simulink model "testModel"  (R2021b)
settings: Solver=FixedStepDiscrete  StartTime=0.0  StopTime=10.0  RelTol=1e-3
libraries: simulink x1
settings Model: DataTypeOverride=Off  Creator=tcollins  LastModifiedBy=imuthi
settings SolverCC: AlgebraicLoopSolver=TrustRegion
settings DataIOCC: LimitDataPoints=on  SaveOutput=off  SaveTime=off  ReturnWorkspaceOutputs=off
settings OptimizationCC: BlockReduction=off  ConditionallyExecuteInputs=off  DefaultParameterBehavior=Inlined  LifeSpan=inf
settings DebuggingCC: AlgebraicLoopMsg=error  SingleTaskRateTransMsg=error  AllowSymbolicDim=off  StrictBusMsg=ErrorOnBusTreatedAsVector  SFUnexpectedBacktrackingDiag=warning  SFNoUnconditionalDefaultTransitionDiag=warning  SFExecutionAtInitializationDiag=none  SFMachineParentedDataDiag=warning  ArithmeticOperatorsInVariantConditions=warning
settings HardwareCC: ProdBitPerPointer=32  ProdBitPerSizeT=32  ProdBitPerPtrDiffT=32  ProdLargestAtomicFloat=None  ProdIntDivRoundTo=Undefined  ProdEndianess=Unspecified  ProdWordSize=32  ProdHWDeviceType=ASIC/FPGA->ASIC/FPGA  ProdEqTarget=off
settings SFSimCC: SimUseLocalCustomCode=off  CustomCodeUndefinedFunction=UseInterfaceOnly
settings RTWCC: RTWUseLocalCustomCode=off
settings CodeAppCC: StateflowObjectComments=on
settings GRTTargetCC: TargetLangStandard=C89/C90 (ANSI)
settings ConfigComp: CovScope=ReferencedModels  CovMetricSettings=dw  CovSaveCumulativeToWorkspaceVar=on  CovSaveSingleToWorkspaceVar=on  CovExternalEMLEnable=off  CovSFcnEnable=off

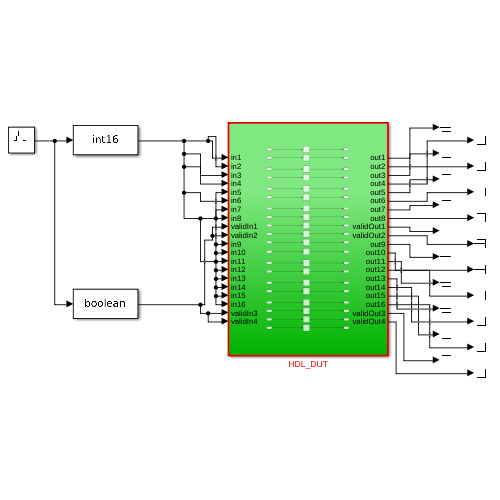
[thumbnail: Simulink's stored preview of the top-level diagram]
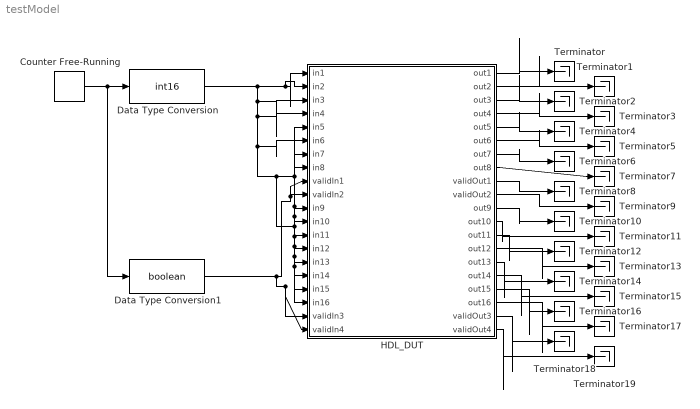
== system testModel ==
  Counter Free-Running : simulink/Sources/Counter Free-Running  NumBits=10  tsamp=1
  Data Type Conversion : DataTypeConversion  OutDataTypeStr=int16
  Data Type Conversion1 : DataTypeConversion  OutDataTypeStr=boolean
  HDL_DUT : Subsystem  TreatAsAtomicUnit=on
  Terminator{,1..19} (20 alike) : Terminator
  wires:
  Counter Free-Running/1 -> Data Type Conversion1/1, Data Type Conversion/1
  HDL_DUT/1(out1) -> Terminator/1
  HDL_DUT/2(out2) -> Terminator1/1
  HDL_DUT/3(out3) -> Terminator2/1
  HDL_DUT/4(out4) -> Terminator3/1
  Data Type Conversion/1 -> HDL_DUT/2(in2), HDL_DUT/1(in1), HDL_DUT/14(in12), HDL_DUT/16(in14), HDL_DUT/18(in16), HDL_DUT/17(in15), HDL_DUT/15(in13), HDL_DUT/11(in9), HDL_DUT/7(in7), HDL_DUT/12(in10), HDL_DUT/13(in11), HDL_DUT/5(in5), HDL_DUT/8(in8), HDL_DUT/6(in6), HDL_DUT/4(in4), HDL_DUT/3(in3)
  HDL_DUT/5(out5) -> Terminator4/1
  HDL_DUT/6(out6) -> Terminator5/1
  HDL_DUT/7(out7) -> Terminator6/1
  HDL_DUT/8(out8) -> Terminator7/1
  Data Type Conversion1/1 -> HDL_DUT/19(validIn3), HDL_DUT/20(validIn4), HDL_DUT/10(validIn2), HDL_DUT/9(validIn1)
  HDL_DUT/9(validOut1) -> Terminator8/1
  HDL_DUT/10(validOut2) -> Terminator9/1
  HDL_DUT/11(out9) -> Terminator10/1
  HDL_DUT/12(out10) -> Terminator11/1
  HDL_DUT/13(out11) -> Terminator12/1
  HDL_DUT/14(out12) -> Terminator13/1
  HDL_DUT/15(out13) -> Terminator14/1
  HDL_DUT/16(out14) -> Terminator15/1
  HDL_DUT/17(out15) -> Terminator16/1
  HDL_DUT/18(out16) -> Terminator17/1
  HDL_DUT/19(validOut3) -> Terminator18/1
  HDL_DUT/20(validOut4) -> Terminator19/1

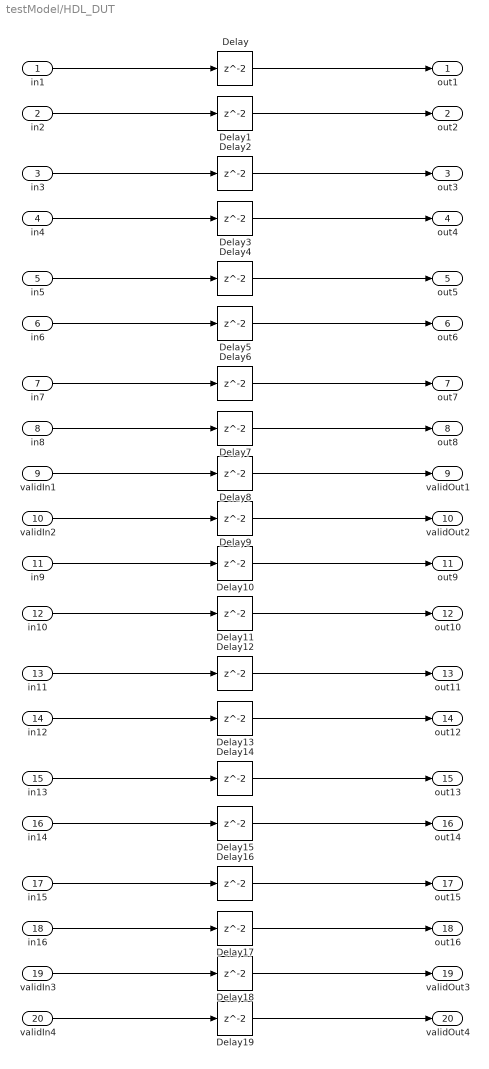
== system testModel/HDL_DUT ==
  in1 : Inport
  in2 : Inport  Port=2
  in3 : Inport  Port=3
  in4 : Inport  Port=4
  in5 : Inport  Port=5
  in6 : Inport  Port=6
  in7 : Inport  Port=7
  in8 : Inport  Port=8
  validIn1 : Inport  Port=9
  validIn2 : Inport  Port=10
  in9 : Inport  Port=11
  in10 : Inport  Port=12
  in11 : Inport  Port=13
  in12 : Inport  Port=14
  in13 : Inport  Port=15
  in14 : Inport  Port=16
  in15 : Inport  Port=17
  in16 : Inport  Port=18
  validIn3 : Inport  Port=19
  validIn4 : Inport  Port=20
  Delay{,1..19} (20 alike) : Delay
  out1 : Outport  VectorParamsAs1DForOutWhenUnconnected=off
  out2 : Outport  Port=2  VectorParamsAs1DForOutWhenUnconnected=off
  out3 : Outport  Port=3  VectorParamsAs1DForOutWhenUnconnected=off
  out4 : Outport  Port=4  VectorParamsAs1DForOutWhenUnconnected=off
  out5 : Outport  Port=5  VectorParamsAs1DForOutWhenUnconnected=off
  out6 : Outport  Port=6  VectorParamsAs1DForOutWhenUnconnected=off
  out7 : Outport  Port=7  VectorParamsAs1DForOutWhenUnconnected=off
  out8 : Outport  Port=8  VectorParamsAs1DForOutWhenUnconnected=off
  validOut1 : Outport  Port=9  VectorParamsAs1DForOutWhenUnconnected=off
  validOut2 : Outport  Port=10  VectorParamsAs1DForOutWhenUnconnected=off
  out9 : Outport  Port=11  VectorParamsAs1DForOutWhenUnconnected=off
  out10 : Outport  Port=12  VectorParamsAs1DForOutWhenUnconnected=off
  out11 : Outport  Port=13  VectorParamsAs1DForOutWhenUnconnected=off
  out12 : Outport  Port=14  VectorParamsAs1DForOutWhenUnconnected=off
  out13 : Outport  Port=15  VectorParamsAs1DForOutWhenUnconnected=off
  out14 : Outport  Port=16  VectorParamsAs1DForOutWhenUnconnected=off
  out15 : Outport  Port=17  VectorParamsAs1DForOutWhenUnconnected=off
  out16 : Outport  Port=18  VectorParamsAs1DForOutWhenUnconnected=off
  validOut3 : Outport  Port=19  VectorParamsAs1DForOutWhenUnconnected=off
  validOut4 : Outport  Port=20  VectorParamsAs1DForOutWhenUnconnected=off
  wires:
  in1/1 -> Delay/1
  Delay/1 -> out1/1
  Delay1/1 -> out2/1
  in2/1 -> Delay1/1
  Delay3/1 -> out4/1
  in3/1 -> Delay2/1
  in4/1 -> Delay3/1
  Delay2/1 -> out3/1
  Delay6/1 -> out7/1
  Delay5/1 -> out6/1
  in7/1 -> Delay6/1
  in8/1 -> Delay7/1
  in5/1 -> Delay4/1
  in6/1 -> Delay5/1
  Delay4/1 -> out5/1
  Delay7/1 -> out8/1
  validIn1/1 -> Delay8/1
  Delay8/1 -> validOut1/1
  Delay9/1 -> validOut2/1
  validIn2/1 -> Delay9/1
  Delay17/1 -> out16/1
  Delay11/1 -> out10/1
  in11/1 -> Delay12/1
  in12/1 -> Delay13/1
  in15/1 -> Delay16/1
  Delay12/1 -> out11/1
  Delay14/1 -> out13/1
  Delay15/1 -> out14/1
  Delay16/1 -> out15/1
  in16/1 -> Delay17/1
  in13/1 -> Delay14/1
  in10/1 -> Delay11/1
  in14/1 -> Delay15/1
  Delay13/1 -> out12/1
  Delay18/1 -> validOut3/1
  validIn3/1 -> Delay18/1
  validIn4/1 -> Delay19/1
  Delay19/1 -> validOut4/1
  Delay10/1 -> out9/1
  in9/1 -> Delay10/1
